simulink model "KinarmUAATask_260120"  (R2019b)
settings: Solver=ode4  StartTime=0.0  StopTime=inf  FixedStep=BKIN_STEP_TIME  RelTol=1e-3  EnableMultiTasking=on
StartFcn:
  |  warndlg('Dexterit-E models cannot run under simulation. Please compile your model and run it from within Dexterit-E.');set_param(bdroot,'SimulationCommand','stop')
model workspace (MAT data in the model file):
  APPROACH_TARGET_COL = 6
  AVOID_TARGET_COL = 2
  BEGIN_TARGET_COL = 3
  BKIN_KINEMATIC_FRAME_SIZE = 400
  BKIN_STEP_TIME = 0.00025
  COLOUR_2ND = 7
  COLOUR_3RD = 11
  COLOUR_4TH = 12
  COLOUR_INIT = 6
  E_APPROACHED = 25
  E_AVOIDED = 23
  E_COND1_APP = 24
  E_COND2_APP = 18
  E_ERROR_TRIAL = 21
  E_FALSE_START = 16
  E_HAND_IN_START = 15
  E_LOC_1 = 1
  E_LOC_10 = 10
  E_LOC_11 = 11
  E_LOC_12 = 12
  E_LOC_2 = 2
  E_LOC_3 = 3
  E_LOC_4 = 4
  E_LOC_5 = 5
  E_LOC_6 = 6
  E_LOC_7 = 7
  E_LOC_8 = 8
  E_LOC_9 = 9
  E_NEUT1_APP = 22
  E_NEUT2_APP = 17
  E_NO_EVENT = 0
  E_SUCCESS_TRIAL = 26
  E_TARGET_ON = 14
  E_TIMED_OUT = 20
  E_TRIAL_COND1 = 27
  E_TRIAL_COND2 = 28
  E_TRIAL_END = 19
  E_TRIAL_NEUT1 = 29
  E_TRIAL_NEUT2 = 30
  E_TRIAL_START = 13
  INFO_TARGET_COL = 5
  LABEL_COL = 4
  LABEL_HEIGHT = 9
  LABEL_TEXT = 8
  LENGTH = 3
  MAX_FORCE = 2
  NEUT_OR_COND = 7
  NUM_SPOTS = 8
  POSTRESP_DELAY = 7
  RADIUS_VIS = 3
  RAMP_DURATION = 3
  REACH_DELAY = 4
  REACH_RAND = 5
  REACH_TO = 6
  START_BLOCK = 9
  START_TARGET_COL = 1
  STROKE_WIDTH = 10
  TARGET_X = 4
  TARGET_Y = 5
  TARG_DIST = 1
  TARG_LENGTH = 3
  TARG_WIDTH = 4
  TOGGLE_FIELD = 8
  WIDTH = 4
  Width = 4
  col_x = 1
  col_y = 2
undefined symbols (not defined in the file or in its folder): slselsubs
libraries: Video x7, General x3, KINARM_general x2, KINARM_EP_loads x2
settings Model: ModifiedComment=chris -- Wed Feb 16 09:18:30 2005 -- Version 1.1384  ModifiedHistory=Feb 16/05 - Add error repeat, add offset ramp  ExtModeArmWhenConnect=off  ExtModeLogAll=off  OrderedModelArguments=off  Creator=Chris Grebeldinger  LastModifiedBy=apark2
settings SolverCC: AutoInsertRateTranBlk=on
settings DataIOCC: SaveFormat=Array  SignalLoggingSaveFormat=ModelDataLogs  SaveOutput=off  SaveTime=off  ReturnWorkspaceOutputs=off  SignalLoggingName=sigsOut
settings OptimizationCC: BlockReduction=off  BooleanDataType=off  OptimizeBlockIOStorage=off  BufferReuse=off  GlobalBufferReuse=off  ExpressionFolding=off  ExpressionDepthLimit=2147483647  LocalBlockOutputs=off  InitFltsAndDblsToZero=on  LifeSpan=inf  OptimizeDataStoreBuffers=off  BusAssignmentInplaceUpdate=off
settings DebuggingCC: SaveWithParameterizedLinksMsg=none  UnderspecifiedInitializationDetection=Classic  MergeDetectMultiDrivingBlocksExec=none  SignalResolutionControl=TryResolveAllWithWarning  MultiTaskDSMMsg=warning  FcnCallInpInsideContextMsg=warning  BusObjectLabelMismatch=none  StateNameClashWarn=warning  StrictBusMsg=ErrorOnBusTreatedAsVector  SFUnexpectedBacktrackingDiag=warning  SFNoUnconditionalDefaultTransitionDiag=warning  SFExecutionAtInitializationDiag=none  ArithmeticOperatorsInVariantConditions=warning
settings HardwareCC: ProdBitPerPointer=32  ProdBitPerSizeT=32  ProdBitPerPtrDiffT=32  ProdLargestAtomicFloat=None  ProdWordSize=32  ProdLongLongMode=on  ProdHWDeviceType=Generic->32-bit x86 compatible  TargetLongLongMode=on  TargetIntDivRoundTo=Zero  TargetEndianess=LittleEndian  TargetHWDeviceType=Generic->32-bit x86 compatible
settings ModelReferenceCC: PropagateSignalLabelsOutOfModel=off
settings SFSimCC: SimCustomHeaderCode="#include \"stdlib.h\""  SimUseLocalCustomCode=off  SimParseCustomCode=off  CustomCodeUndefinedFunction=UseInterfaceOnly
settings RTWCC: Description=Simulink Real-Time  SystemTargetFile=slrt.tlc  TemplateMakefile=slrt_default_tmf  RTWUseLocalCustomCode=off  CustomSourceCode="#include \"stdlib.h\""  CodeExecutionProfiling=on
settings CodeAppCC: MaxIdLength=63  StateflowObjectComments=on
settings SimulinkRealTimeCC: TargetFcnLib=ansi_tfl_tmw.mat  GeneratePreprocessorConditionals=Disable all  PreserveStateflowLocalDataDimensions=off
settings ConfigComp: CovMetricSettings=dw  CovHtmlReporting=on  CovSaveCumulativeToWorkspaceVar=on  CovSaveSingleToWorkspaceVar=on  CovExternalEMLEnable=off

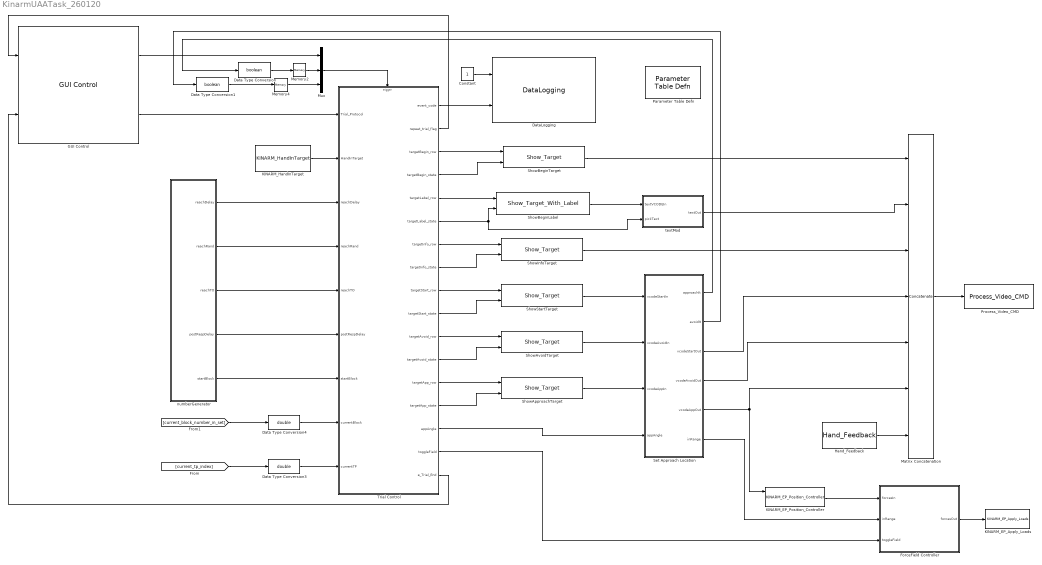
== system KinarmUAATask_260120 ==
  Constant : Constant
  Data Type Conversion : DataTypeConversion  OutDataTypeStr=boolean
  Data Type Conversion1 : DataTypeConversion  OutDataTypeStr=boolean
  Data Type Conversion3 : DataTypeConversion  OutDataTypeStr=double
  Data Type Conversion4 : DataTypeConversion  OutDataTypeStr=double
  DataLogging : General/DataLogging  log_event_codes=on  log_analog_inputs=off  show_time_remaining=off  ecat_include=on
  ForceField Controller : Subsystem
  GUI Control : General/GUI Control  task_version=1.0  show_repeat_trial_flag=on  use_custom_tp=off  target_type_str=Circle  Target_Type=1  XYcols=[1 2]  Vcols=3  Lcols=4  indices_padding=[0 0 0 0;0 0 0 0]  target_table_rows=64  load_table_rows=20  tp_table_rows=100
  Hand_Feedback : KINARM_general/Hand_Feedback  feedback_cntl_src=none
  KINARM_EP_Apply_Loads : KINARM_EP_loads/KINARM_EP_Apply_Loads  up_duration=1500  down_duration=1500  max_force=30
  KINARM_EP_Position_Controller : KINARM_EP_loads/KINARM_EP_Position_Controller  use_dom_hand=on  inertias_for_FF=KINARM End Point robot  gain_choice=Standard Movement  sample_time=0.001
  KINARM_HandInTarget : KINARM_general/KINARM_HandInTarget  use_dominant_hand=on  target_type=Circle  num_states=1  attribcol1=[RADIUS_VIS]  attribcol2=[0]  attribcol3=[0]  attribcol4=[0]  attribcol5=[0]
  Matrix Concatenation : Concatenate  NumInputs=7  Mode=Multidimensional array
  Memory2 : Memory
  Memory4 : Memory
  Mux : Mux  Inputs=3
  Parameter Table Defn : General/Parameter Table Defn  ShowInLibBrowser=0
  Process_Video_CMD : Video/Process_Video_CMD  video_delay=50
  Set Approach Location : Subsystem
  ShowApproachTarget : Video/Show_Target  target_type=Circle  num_states=1  attribcol1=[COLOUR_INIT 0 0 RADIUS_VIS]  attribcol2=[0 0 0 0]  attribcol3=[0 0 0 0]  attribcol4=[0 0 0 0]  attribcol5=[0 0 0 0]  stateindices_padding=[0 0 0 0 0 0 0;0 0 0 0 0 0 0;0 0 0 0 0 0 0;0 0 0 0 0 0 0;0 0 0 0 0 0 0]  source=dialog  opacity=100  target_display=Both subject and operator displays  num_col=4
  ShowAvoidTarget : Video/Show_Target  target_type=Circle  num_states=1  attribcol1=[COLOUR_INIT COLOUR_2ND STROKE_WIDTH RADIUS_VIS]  attribcol2=[0 0 0 0]  attribcol3=[0 0 0 0]  attribcol4=[0 0 0 0]  attribcol5=[0 0 0 0]  stateindices_padding=[0 0 0 0 0 0 0;0 0 0 0 0 0 0;0 0 0 0 0 0 0;0 0 0 0 0 0 0;0 0 0 0 0 0 0]  source=dialog  opacity=100  target_display=Both subject and operator displays  num_col=4
  ShowBeginLabel : Video/Show_Target_With_Label  target_type=Circle  num_states=3  attribcol1=[0 0 0 0 LABEL_TEXT COLOUR_INIT LABEL_HEIGHT]  attribcol2=[0 0 0 0 LABEL_TEXT COLOUR_2ND LABEL_HEIGHT]  attribcol3=[0 0 0 0 LABEL_TEXT COLOUR_3RD LABEL_HEIGHT]  attribcol4=[0 0 0 0 0 0 0]  attribcol5=[0 0 0 0 0 0 0]  stateindices_padding=[0 0 0 0;0 0 0 0;0 0 0 0;0 0 0 0;0 0 0 0]  source=dialog  opacity=100  target_display=Both subject and operator displays
  ShowBeginTarget : Video/Show_Target  target_type=Circle  num_states=1  attribcol1=[COLOUR_INIT COLOUR_2ND STROKE_WIDTH RADIUS_VIS]  attribcol2=[0 0 0 0]  attribcol3=[0 0 0 0]  attribcol4=[0 0 0 0]  attribcol5=[0 0 0 0]  stateindices_padding=[0 0 0 0 0 0 0;0 0 0 0 0 0 0;0 0 0 0 0 0 0;0 0 0 0 0 0 0;0 0 0 0 0 0 0]  source=dialog  opacity=100  target_display=Both subject and operator displays  num_col=4
  ShowInfoTarget : Video/Show_Target  target_type=Rectangle  num_states=4  attribcol1=[COLOUR_INIT 0 0 TARGET_X TARGET_Y 0]  attribcol2=[COLOUR_2ND 0 0 TARGET_X TARGET_Y 0]  attribcol3=[COLOUR_3RD 0 0 TARGET_X TARGET_Y 0]  attribcol4=[COLOUR_4TH 0 0 TARGET_X TARGET_Y 0]  attribcol5=[0 0 0 0 0 0]  stateindices_padding=[0 0 0 0 0;0 0 0 0 0;0 0 0 0 0;0 0 0 0 0;0 0 0 0 0]  source=dialog  opacity=100  target_display=Both subject and operator displays  num_col=6
  ShowStartTarget : Video/Show_Target  target_type=Circle  num_states=1  attribcol1=[COLOUR_INIT COLOUR_2ND STROKE_WIDTH RADIUS_VIS]  attribcol2=[0 0 0 0]  attribcol3=[0 0 0 0]  attribcol4=[0 0 0 0]  attribcol5=[0 0 0 0]  stateindices_padding=[0 0 0 0 0 0 0;0 0 0 0 0 0 0;0 0 0 0 0 0 0;0 0 0 0 0 0 0;0 0 0 0 0 0 0]  source=dialog  opacity=100  target_display=Both subject and operator displays  num_col=4
  Trial Control : Stateflow chart  TreatAsAtomicUnit=on
  numberGenerator : Subsystem
  textMod : Subsystem
  wires:
  Trial Control/17(e_Trial_End) -> GUI Control/2
  Trial Control/10(targetStart_state) -> ShowStartTarget/2
  Trial Control/9(targetStart_row) -> ShowStartTarget/1
  Matrix Concatenation/1 -> Process_Video_CMD/1
  Trial Control/1(event_code) -> DataLogging/2
  ShowStartTarget/1 -> Set Approach Location/1(vcodeStartIn)
  Constant/1 -> DataLogging/1
  GUI Control/2 -> Trial Control/1(Trial_Protocol)
  Trial Control/13(targetApp_row) -> ShowApproachTarget/1
  Trial Control/14(targetApp_state) -> ShowApproachTarget/2
  Trial Control/2(repeat_trial_flag) -> GUI Control/1
  KINARM_EP_Position_Controller/1 -> ForceField Controller/1(forcesIn)
  [current_tp_index] -> Data Type Conversion3/1
  ShowApproachTarget/1 -> Set Approach Location/3(vcodeAppIn)
  Set Approach Location/5(vcodeAppOut) -> Matrix Concatenation/6, KINARM_EP_Position_Controller/1
  Trial Control/15(appAngle) -> Set Approach Location/4(appAngle)
  ShowInfoTarget/1 -> Matrix Concatenation/3
  KINARM_HandInTarget/1 -> Trial Control/2(HandInTarget)
  Trial Control/16(toggleField) -> ForceField Controller/3(toggleField)
  ForceField Controller/1(forcesOut) -> KINARM_EP_Apply_Loads/1
  Trial Control/3(targetBegin_row) -> ShowBeginTarget/1
  Trial Control/4(targetBegin_state) -> ShowBeginTarget/2
  Trial Control/7(targetInfo_row) -> ShowInfoTarget/1
  Trial Control/8(targetInfo_state) -> ShowInfoTarget/2
  Trial Control/5(targetLabel_row) -> ShowBeginLabel/1
  Trial Control/6(targetLabel_state) -> ShowBeginLabel/2, textMod/2(pickText)
  numberGenerator/1(reachDelay) -> Trial Control/3(reachDelay)
  numberGenerator/2(reachRand) -> Trial Control/4(reachRand)
  numberGenerator/3(reachTO) -> Trial Control/5(reachTO)
  numberGenerator/4(postRespDelay) -> Trial Control/6(postRespDelay)
  ShowBeginLabel/1 -> textMod/1(textVCODEIn)
  ShowBeginTarget/1 -> Matrix Concatenation/1
  Hand_Feedback/1 -> Matrix Concatenation/7
  Set Approach Location/6(inRange) -> ForceField Controller/2(inRange)
  Data Type Conversion3/1 -> Trial Control/9(currentTP)
  Trial Control/11(targetAvoid_row) -> ShowAvoidTarget/1
  Trial Control/12(targetAvoid_state) -> ShowAvoidTarget/2
  ShowAvoidTarget/1 -> Set Approach Location/2(vcodeAvoidIn)
  [current_block_number_in_set] -> Data Type Conversion4/1
  Data Type Conversion4/1 -> Trial Control/8(currentBlock)
  textMod/1(textOut) -> Matrix Concatenation/2
  Data Type Conversion1/1 -> Memory4/1
  Memory4/1 -> Mux/3
  Data Type Conversion/1 -> Memory2/1
  Memory2/1 -> Mux/2
  Mux/1 -> Trial Control/Trigger
  GUI Control/1 -> Mux/1
  Set Approach Location/1(approachIt) -> Data Type Conversion/1
  Set Approach Location/4(vcodeAvoidOut) -> Matrix Concatenation/5
  Set Approach Location/2(avoidIt) -> Data Type Conversion1/1
  Set Approach Location/3(vcodeStartOut) -> Matrix Concatenation/4
  numberGenerator/5(startBlock) -> Trial Control/7(startBlock)

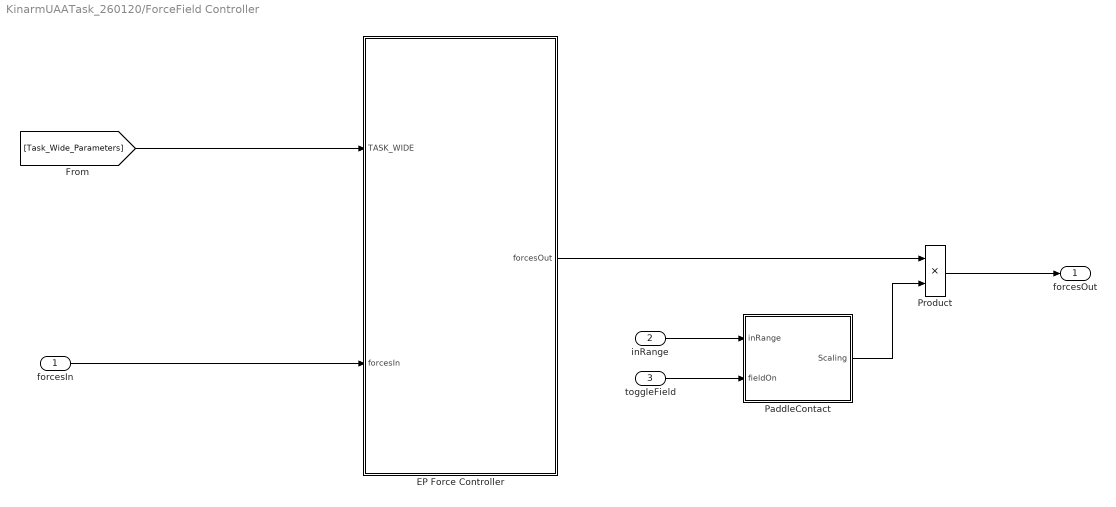
== system KinarmUAATask_260120/ForceField Controller ==
  forcesIn : Inport
  inRange : Inport  Port=2
  toggleField : Inport  Port=3
  EP Force Controller : MATLAB Function  TreatAsAtomicUnit=on
  PaddleContact : Subsystem  mask(Perturbation){}
  Product : Product
  forcesOut : Outport
  wires:
  [Task_Wide_Parameters] -> EP Force Controller/1(TASK_WIDE)
  EP Force Controller/1(forcesOut) -> Product/1
  toggleField/1 -> PaddleContact/2(fieldOn)
  forcesIn/1 -> EP Force Controller/2(forcesIn)
  PaddleContact/1(Scaling) -> Product/2
  inRange/1 -> PaddleContact/1(inRange)
  Product/1 -> forcesOut/1

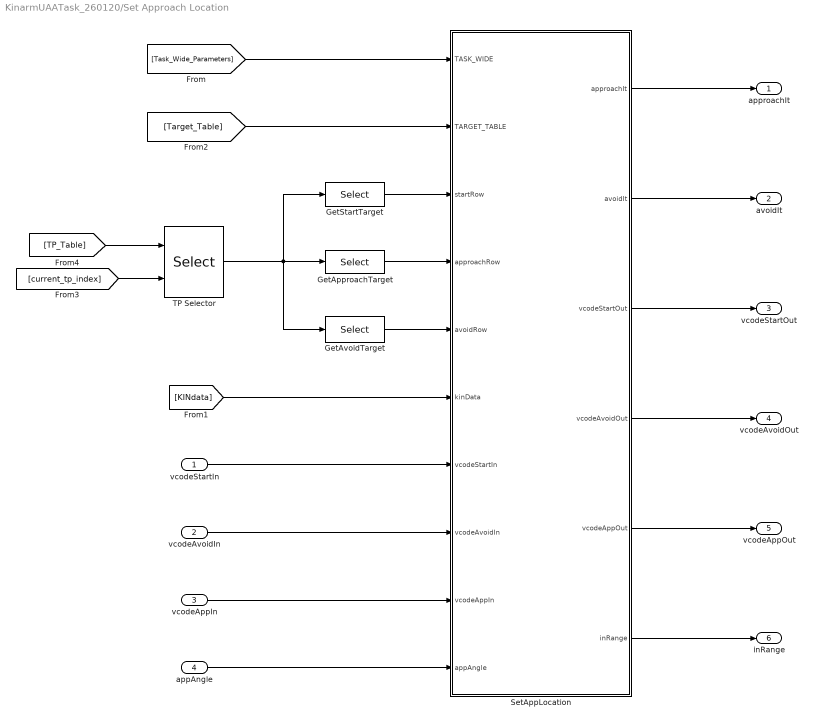
== system KinarmUAATask_260120/Set Approach Location ==
  vcodeStartIn : Inport
  vcodeAvoidIn : Inport  Port=2
  vcodeAppIn : Inport  Port=3
  appAngle : Inport  Port=4
  GetApproachTarget : Selector  NumberOfDimensions=2  InputPortWidth=3  IndexOptions=Select all,Index vector (dialog)  Indices=[1],[APPROACH_TARGET_COL]  OutputSizes=slselsubs([(-2),(-2)],1),slselsubs([(-2),(-2)],2)
  GetAvoidTarget : Selector  NumberOfDimensions=2  InputPortWidth=3  IndexOptions=Select all,Index vector (dialog)  Indices=[1],[AVOID_TARGET_COL]  OutputSizes=slselsubs([(-2),(-2)],1),slselsubs([(-2),(-2)],2)
  GetStartTarget : Selector  NumberOfDimensions=2  InputPortWidth=3  IndexOptions=Select all,Index vector (dialog)  Indices=[1],[START_TARGET_COL]  OutputSizes=slselsubs([(-2),(-2)],1),slselsubs([(-2),(-2)],2)
  SetAppLocation : MATLAB Function  TreatAsAtomicUnit=on
  TP Selector : Selector  NumberOfDimensions=2  InputPortWidth=3  IndexOptions=Index vector (port),Select all  Indices=1,-1  OutputSizes=slselsubs([(-2),(-2)],1),slselsubs([(-2),(-2)],2)
  approachIt : Outport
  avoidIt : Outport  Port=2
  vcodeStartOut : Outport  Port=3
  vcodeAvoidOut : Outport  Port=4
  vcodeAppOut : Outport  Port=5
  inRange : Outport  Port=6
  wires:
  [Task_Wide_Parameters] -> SetAppLocation/1(TASK_WIDE)
  [current_tp_index] -> TP Selector/2
  [KINdata] -> SetAppLocation/6(kinData)
  [TP_Table] -> TP Selector/1
  [Target_Table] -> SetAppLocation/2(TARGET_TABLE)
  vcodeAppIn/1 -> SetAppLocation/9(vcodeAppIn)
  SetAppLocation/5(vcodeAppOut) -> vcodeAppOut/1
  GetStartTarget/1 -> SetAppLocation/3(startRow)
  appAngle/1 -> SetAppLocation/10(appAngle)
  SetAppLocation/6(inRange) -> inRange/1
  vcodeAvoidIn/1 -> SetAppLocation/8(vcodeAvoidIn)
  GetAvoidTarget/1 -> SetAppLocation/5(avoidRow)
  GetApproachTarget/1 -> SetAppLocation/4(approachRow)
  TP Selector/1 -> GetStartTarget/1, GetAvoidTarget/1, GetApproachTarget/1
  SetAppLocation/4(vcodeAvoidOut) -> vcodeAvoidOut/1
  SetAppLocation/1(approachIt) -> approachIt/1
  SetAppLocation/2(avoidIt) -> avoidIt/1
  vcodeStartIn/1 -> SetAppLocation/7(vcodeStartIn)
  SetAppLocation/3(vcodeStartOut) -> vcodeStartOut/1

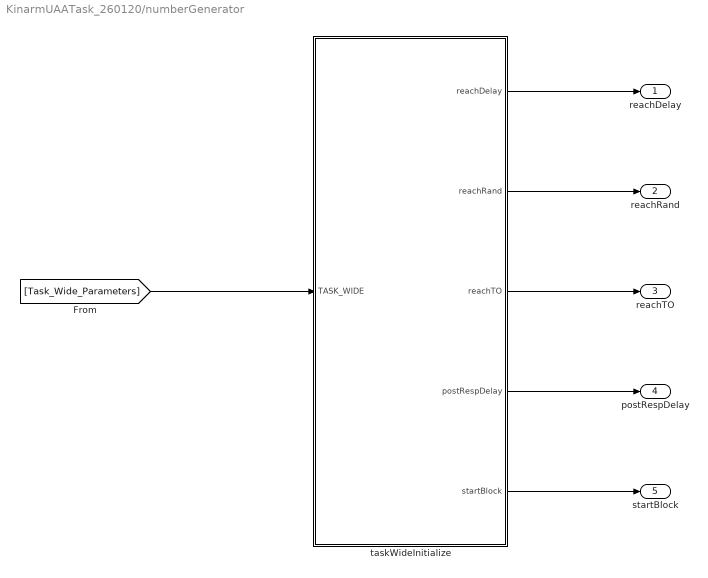
== system KinarmUAATask_260120/numberGenerator ==
  taskWideInitialize : MATLAB Function  TreatAsAtomicUnit=on
  reachDelay : Outport
  reachRand : Outport  Port=2
  reachTO : Outport  Port=3
  postRespDelay : Outport  Port=4
  startBlock : Outport  Port=5
  wires:
  [Task_Wide_Parameters] -> taskWideInitialize/1(TASK_WIDE)
  taskWideInitialize/1(reachDelay) -> reachDelay/1
  taskWideInitialize/2(reachRand) -> reachRand/1
  taskWideInitialize/3(reachTO) -> reachTO/1
  taskWideInitialize/4(postRespDelay) -> postRespDelay/1
  taskWideInitialize/5(startBlock) -> startBlock/1

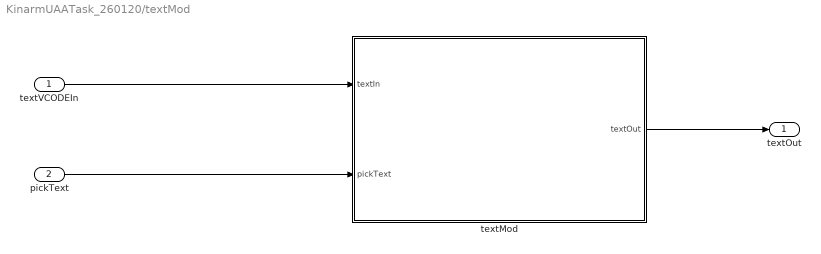
== system KinarmUAATask_260120/textMod ==
  textVCODEIn : Inport
  pickText : Inport  Port=2
  textMod : MATLAB Function  TreatAsAtomicUnit=on
  textOut : Outport
  wires:
  textMod/1(textOut) -> textOut/1
  textVCODEIn/1 -> textMod/1(textIn)
  pickText/1 -> textMod/2(pickText)

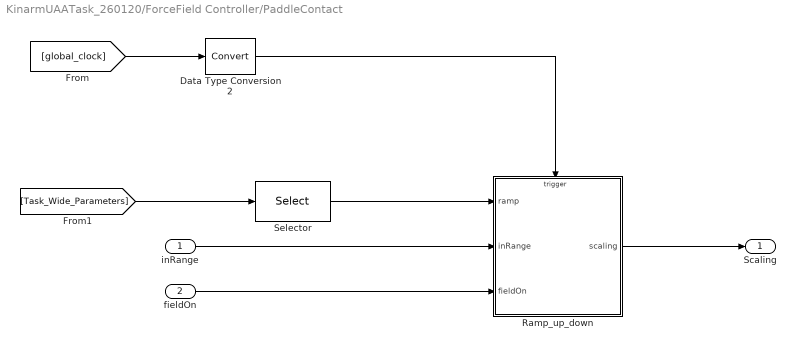
== system KinarmUAATask_260120/ForceField Controller/PaddleContact ==
  inRange : Inport
  fieldOn : Inport  Port=2
  Data Type Conversion2 : DataTypeConversion
  Ramp_up_down : Stateflow chart  TreatAsAtomicUnit=on
  Selector : Selector  NumberOfDimensions=2  InputPortWidth=3  IndexOptions=Index vector (dialog),Select all  Indices=[RAMP_DURATION],[3]  OutputSizes=slselsubs([(-2),(-2)],1),1
  Scaling : Outport
  wires:
  Ramp_up_down/1(scaling) -> Scaling/1
  [global_clock] -> Data Type Conversion2/1
  Data Type Conversion2/1 -> Ramp_up_down/Trigger
  [Task_Wide_Parameters] -> Selector/1
  Selector/1 -> Ramp_up_down/1(ramp)
  inRange/1 -> Ramp_up_down/2(inRange)
  fieldOn/1 -> Ramp_up_down/3(fieldOn)

== matlab function KinarmUAATask_260120/Set Approach Location/SetAppLocation ==
  data: approachIt output; avoidIt output; vcodeStartOut output; vcodeAvoidOut output; vcodeAppOut output; TASK_WIDE input; TARGET_TABLE input; startRow input; approachRow input; avoidRow input; kinData input; vcodeStartIn input; vcodeAvoidIn input; vcodeAppIn input; appAngle input; TARG_DIST parameter; RADIUS_VIS parameter; inRange output; NUM_SPOTS parameter
function [approachIt, avoidIt, vcodeStartOut, vcodeAvoidOut, vcodeAppOut, inRange] = fcn...
    (TASK_WIDE, TARGET_TABLE, startRow, approachRow, avoidRow, kinData, vcodeStartIn, vcodeAvoidIn, vcodeAppIn, appAngle,...
    TARG_DIST, RADIUS_VIS, NUM_SPOTS)
%This function checks if the hand is in the approach or avoid targets and passing through the start target for nice visuals.

%% initialize hand and location to be displayed
targDist = TASK_WIDE(TARG_DIST)*0.01; %gets distance of targets set from task wide
numSpots = TASK_WIDE(NUM_SPOTS); %get the number of reach spots but still needs a change in the Trial Control to align with the maximum appAngle
angleArray = [0:2*pi/numSpots:2*pi-2*pi/numSpots]; %get radians for each location

whichLoc = angleArray(appAngle); %get the location

%% initialize radius
vcodeStartOut = vcodeStartIn; %start target routed through this function
rValStart = TARGET_TABLE(startRow,RADIUS_VIS)*0.01; %radius of start target
rValApp = TARGET_TABLE(approachRow,RADIUS_VIS)*0.01; %radius of approach target
rValApp2 = targDist-rValStart; %radius of force field around approach target accounts for starting target
rValAvoid = TARGET_TABLE(avoidRow,RADIUS_VIS)*0.01; %radius of avoid target

asseHand=kinData(3,1); %check which hand is used
handX = kinData(asseHand,23); %get the x position of the hand
handY = kinData(asseHand,24); %get the y position of the hand

%% change vcodes for approach target contact
%Rip off of handintarget function for a shifted approach target (circle).
vcodeAppOut = vcodeAppIn;

vcodeAppOut(3) = vcodeStartIn(3) + targDist*cos(whichLoc); %get shifted x position of the approach target
vcodeAppOut(4) = vcodeStartIn(4) + targDist*sin(whichLoc); %get shifted y position of the approach target

deltaxApp=handX-vcodeAppOut(3); %get the difference between hand x position and approach target x position
deltayApp=handY-vcodeAppOut(4); %get the difference between hand y position and approach target y position

distanceApp = deltaxApp.^2 + deltayApp.^2; %get the hypotenuse squared
if (distanceApp < rValApp^2) %if hand inside approach target
    approachIt = 1; %flag is 1
else
    approachIt = 0; %flag is 0
end

%if hand inside the force field, won't turn on forcefield unless
%toggleField = 1 in Trial Control
if (distanceApp < rValApp2^2) %check if hand is within forcefield
    inRange = 1; %flag is 1
else
    inRange = 0; %flag is 0
end

%% change vcodes for avoid target no contact
%similar to above but checks if hand is inside avoid target (circle)

vcodeAvoidOut = vcodeAvoidIn;

vcodeAvoidOut(3) = vcodeStartIn(3) + targDist*cos(whichLoc+pi); %shifted x position of avoid target
vcodeAvoidOut(4) = vcodeStartIn(4) + targDist*sin(whichLoc+pi);

deltaxAvoid=handX-vcodeAvoidOut(3);
deltayAvoid=handY-vcodeAvoidOut(4);

distanceAvoid = deltaxAvoid.^2 + deltayAvoid.^2;
if (distanceAvoid < rValAvoid^2) %if hand inside approach target
    avoidIt = 1;
else
    avoidIt = 0;
end

== stateflow chart KinarmUAATask_260120/Trial Control ==
  note: ************************Preface***************************:
      | The UKA task examines approach and avoidance tendencies to certain visual stimulus shown to participants. Typically, two conditions are used and testing by having participants remember
      | to approach one condition and avoid the other (move in the opposite direction). This is done in one block and the association is reverse in the next block.
      | Previous approach and avoidance tasks AAT used keyboard presses or joysticks to examine these tendencies but were biased by testing only unimanual movements.
      |
      | This adaptation of the AAT examines tendencies in 12 different directions where 1 is east of the start target, 4 is north, 7 is west, and 10 is south.
      | This version has neutral conditions that compares baseline movements to neutral stimulus resulting in 4 different types of images.
      | The current .dtp file uses 6 different images of condition1 and 6 images of condition2 stimulus and 6 neutral images based on the shape of the condition1 images and 6 neutral images
      | based on the shape of the condition2 images. Each image is associated with a specific TP so there are 24 total TP to call. TP1-6 are condition1 images, 7-12 are condition2 images,
      | 13-18 are neutral condition1 images, 19-24 are neutral condition2 images.
      |
      | The task is set up so that each block only consists of conditions or neutral images so each block has only TP1-12 or TP13-24. In each of these blocks, each condition or neutral image
      | appears in each of the 12 directions at least once (i.e. in a condition block, TP1-6 appears in locations 1-12 at least once and TP7-12 appears at least once so each set of 6TP needs
      | to be run twice as a group of 24 trials for an even distribution of conditions/reach direction).
      |
      | The task must be run in 4 blocks starting and ending with a condition or neutral block, and the middle two blocks being the other block type for proper task operation. The UKA
      | randomly selects which condition will first be associated with approach and avoidance but when the next block of the same condition appears, the association is automatically
      | reversed (neutCount == 1 or condCount == 1).
      |
      | *This layout assumes the task has 12 directions of reach and 6images per 4conditions to run properly
      | *Modifying the task to have less reach directions, less images in the TP, or a different number of blocks requires testing
      | *approaching a condition also equals avoiding the other within each block
  state Initialize/
    %set up targets and states
    entry:
    targetInfo_row = Trial_Protocol(INFO_TARGET_COL); %image of approach/avoid association
    targetBegin_row = Trial_Protocol(BEGIN_TARGET_COL); %block start target
    targetStart_row = Trial_Protocol(START_TARGET_COL); %trial start target
    targetApp_row = Trial_Protocol(APPROACH_TARGET_COL); %approach target
    targetAvoid_row = Trial_Protocol(AVOID_TARGET_COL); %avoid target
    targetLabel_row = Trial_Protocol(LABEL_COL); %target for displaying text
    targetInfo_state = 0; %turn off information target
    targetBegin_state = 0; %turn off block start trial
    targetStart_state = 0; %turn off trial start target
    targetApp_state = 0; %turn off approach target
    targetAvoid_state = 0; %turn off avoid target
    targetLabel_state = 0; %turn off label
  state MainTrial/
    state StartofTrial/
      %start trial
      entry:
      targetApp_row = Trial_Protocol(APPROACH_TARGET_COL); %approach target
      targetAvoid_row = Trial_Protocol(AVOID_TARGET_COL); %avoid target
      randReach = reachRand*rand(); %get random value for reachRand
      targetStart_state = 1; %show start trial target
      targetApp_state = 0; %turn off approach target
      targetAvoid_state = 0; %turn off avoid target
      toggleField = 0; %no forcefield also doubles as indicating cond2/neut2 targets
      targetBegin_state = 0; %turn off start task target
      targetLabel_state = 0; %turn off labels
      targetInfo_state = 0; %turn off info target
      countTP(currentTP) = countTP(currentTP) + 1; %increment the countTP at the currentTP index
      [appAngle, condNeut] = arraySets(randA,randB,countTP,currentTP); %function to get random location
      event_code = E_TRIAL_START; %trial started
    state condEvents/
      state approachCond1/
        event_code = E_COND1_APP;
        targetInfo_state = 1; %turn on info
      state approachCond2/
        event_code = E_COND2_APP;
        targetInfo_state = 2; %turn on info
    state waitForHold/
    state outputBlockOrder/
      %set up approach or avoid for condition and neutral trials based on even or odd of the current trial
      entry:
      appAvoidCond = mod(currentTP,2); %even is approach cond1/avoid cond2, odd is approach cond2/avoid cond1
      appAvoidNeut = mod(currentTP,2); %same as condition block
      condCount = 0; %count the condition blocks
      neutCount = 0; %count the neutral blocks
    state condCount/
      %sets the condition block
      entry:
      condCount = condCount + 1; %increment condition block
      appAvoid = appAvoidCond; %set approach/avoid
    state blockStart/
      %get the current block number and set up TP counter
      %and randA for random order for cond1/neut1 and
      %randB for cont2/neut2. Not sure how to make
      %randperm take Task_Wide input
      entry:
      blockCheck = currentBlock; %update blockNumber
      targetBegin_state = 1; %turn on task start target
      targetLabel_state = 1; %turn on label target
      countTP = zeros(1,24); %set TP count
      randA = randperm(12); %set rand array of locations
      randB = randperm(12); %set rand array of locations
    state handStart/
      %participant reads
      %instructions so wait for
      %the hand to be in start
      %target for some time
    state left/
      %event code for hand leaving start
      event_code = E_FALSE_START;
    state AppOn/
      %turn on targets for reaching
      entry:
      toggleField = Trial_Protocol(TOGGLE_FIELD); %check if trial
      %has forcefield turns on a forcefield if it is set but also just
      %indicates that a trial is cond1/neut1 (1) or cond2/neut2 (2)
      targetStart_state = 0; %turn off start target
      targetApp_state = 1; %turn on approach target
      targetAvoid_state = 1; %turn on avoid target
    state swapNeutBlock/
      %swap the approach avoid rule
      entry:
      appAvoidNeut = 1-appAvoidNeut;
    state neutCount/
      %sets the neutral block
      entry:
      neutCount = neutCount + 1; %increment neutral block
      appAvoid = appAvoidNeut; %set approach from current block type
    state whichSide/
      %the hand is in the start target
      event_code = E_HAND_IN_START;
    state conditionEvents
      state eventCond1/
        event_code = E_TRIAL_COND1;
      state eventCond2/
        event_code = E_TRIAL_COND2;
      state eventNeut1/
        event_code = E_TRIAL_NEUT1;
      state eventNeut2/
        event_code = E_TRIAL_NEUT2;
    state swapCondBlock/
      %swap the approach avoid condition
      entry:
      appAvoidCond = 1-appAvoidCond;
    state neutEvents/
      state approachNeut1/
        event_code = E_NEUT1_APP;
        targetInfo_state = 3; %turn on info
      state approachNeut2/
        event_code = E_NEUT2_APP;
        targetInfo_state = 4; %turn on info
    state nice1/
    state waitForHold1/
    state nice/
    state Approached/
      %hand is in approach
      event_code = E_APPROACHED;
      toggleField = 0; %turn off forcefield
    state locationEvents/
      state loc1/
        event_code = E_LOC_1;
      state loc2/
        event_code = E_LOC_2;
      state loc3/
        event_code = E_LOC_3;
      state loc4/
        event_code = E_LOC_4;
      state loc5/
        event_code = E_LOC_5;
      state loc6/
        event_code = E_LOC_6;
      state loc7/
        event_code = E_LOC_7;
      state loc8/
        event_code = E_LOC_8;
      state loc9/
        event_code = E_LOC_9;
      state loc10/
        event_code = E_LOC_10;
      state loc11/
        event_code = E_LOC_11;
      state loc12/
        event_code = E_LOC_12;
    state checkError/
      %trial was error
      event_code = E_ERROR_TRIAL;
      targetLabel_state = 2; %incorrect!
    state Avoided/
      %hand left avoid target
      event_code = E_AVOIDED;
      toggleField = 0; %turn off forcefield
    state success/
      %trial was successful
      event_code = E_SUCCESS_TRIAL;
    state EndOfTrial/
      % Turn off targets,
      targetStart_state = 0; %turn off start target
      targetAvoid_state = 0; %turn off avoid target
      targetApp_state = 0; %turn off approach target
      toggleField = 0; %turn off forcefield
    state TimedOut/
      %too slow to reach start/app/avoid
      event_code = E_TIMED_OUT;
      targetLabel_state = 3; %too slow!
      toggleField = 0; %turn off forcefield
    condEvents -> waitForHold : after(1,msec)
    condCount -> approachCond1 [order 1] : %approach cond1
        | [appAvoid == 0]
    waitForHold -> handStart : %hand in
        | [HandInTarget(targetBegin_row) == 1]
    handStart -> waitForHold [order 2] : %hand out
        | [HandInTarget(targetBegin_row) == 0]
    (junction 357) -> outputBlockOrder [order 2] : %if second neut block finished
        | [neutCount == 2]
    (junction 355) -> outputBlockOrder [order 2] : %if second cond block finished
        | [condCount == 2]
    outputBlockOrder -> blockStart : %start task
    condCount -> approachCond2 [order 2] : %approach cond2
        | [appAvoid == 1]
    handStart -> StartofTrial [order 3] : %hand in start target for long enough
        | after(startBlock,msec)
    StartofTrial -> (junction 455)
    blockStart -> condCount [order 1] : %if condition block
        | [Trial_Protocol(NEUT_OR_COND) == 1]
    (junction 357) -> blockStart [order 1] : %if no neut block started
        | [neutCount == 0]
    (junction 357) -> swapNeutBlock [order 3] : %if first neut block finished
        | [neutCount == 1]
    waitForHold1 -> handStart : %hand in
        | [HandInTarget(targetBegin_row) == 1]
    handStart -> waitForHold1 [order 1] : %hand out
        | [HandInTarget(targetBegin_row) == 0]
    (junction 323) -> (junction 357) [order 2] : %if neutral block
        | [Trial_Protocol(NEUT_OR_COND) == 0]
    left -> (junction 455) : %after a time
        | after(postRespDelay/2,msec)
    (junction 455) -> whichSide : %checks if hand is in start
        | [HandInTarget(targetStart_row) == 1]
    whichSide -> left [order 1] : %check if hand left start
        | [HandInTarget(targetStart_row) == 0]
    blockStart -> neutCount [order 2] : %if neutral block
        | [Trial_Protocol(NEUT_OR_COND) == 0]
    swapNeutBlock -> blockStart
    (junction 355) -> blockStart [order 1] : %if no cond block started
        | [condCount == 0]
    swapCondBlock -> blockStart
    whichSide -> AppOn [order 2] : %hand in start delay
        | after(reachDelay+randReach,msec)
    neutCount -> approachNeut2 [order 1] : %approach neut2
        | [appAvoid == 1]
    neutCount -> approachNeut1 [order 2] : %approach neut1
        | [appAvoid == 0]
    AppOn -> eventCond1 [order 2] : %condition1
        | [condNeut == 1]
    AppOn -> eventCond2 [order 3] : %condition 2
        | [condNeut == 2]
    AppOn -> eventNeut1 [order 4] : %neutral 1
        | [condNeut == 3]
    AppOn -> eventNeut2 [order 1] : %neutral 2
        | [condNeut == 4]
    (junction 323) -> (junction 355) [order 1] : %if condition block
        | [Trial_Protocol(NEUT_OR_COND) == 1]
    (junction 355) -> swapCondBlock [order 3] : %if first cond block finished
        | [condCount == 1]
    neutEvents -> waitForHold1 : after(1,msec)
    conditionEvents -> nice1 : after(1,msec)
    Approached -> nice [order 1] : %approached cond2/neut2 during approach cond1/neut1 block
        | [(Trial_Protocol(TOGGLE_FIELD) == 1) && appAvoid == 0]
    Approached -> nice [order 2] : %approached cond1/neut1 during approach cond2/neut2 block
        | [(Trial_Protocol(TOGGLE_FIELD) == 0) && appAvoid == 1]
    locationEvents -> Approached [order 2] : %check if approached
        | e_approach
    nice -> checkError : after(1,msec)
    Approached -> success [order 3] : after(1,msec)
    nice1 -> loc1 [order 1] : %check where the
        | %target is
        | [appAngle == 1]
    nice1 -> loc2 [order 2] : [appAngle == 2]
    Avoided -> nice [order 1] : %avoided cond2/neut2 during an approach cond2/neut2 block
        | [(Trial_Protocol(TOGGLE_FIELD) == 1) && appAvoid == 1]
    checkError -> EndOfTrial : %delay after error trial
        | after(postRespDelay,msec)
    nice1 -> loc3 [order 3] : [appAngle == 3]
    locationEvents -> Avoided [order 3] : %check if avoided
        | e_avoid
    Avoided -> nice [order 2] : %avoided cond1/neut1 during an approach cond1/neut1 block
        | [(Trial_Protocol(TOGGLE_FIELD) == 0) && appAvoid == 0]
    nice1 -> loc4 [order 4] : [appAngle == 4]
    nice1 -> loc5 [order 5] : [appAngle == 5]
    Avoided -> success [order 3] : after(1,msec)
    nice1 -> loc6 [order 6] : [appAngle == 6]
    nice1 -> loc7 [order 7] : [appAngle == 7]
    nice1 -> loc8 [order 8] : [appAngle == 8]
    success -> EndOfTrial : %delay for success
        | after(postRespDelay,msec)
    nice1 -> loc9 [order 9] : [appAngle == 9]
    nice1 -> loc10 [order 10] : [appAngle == 10]
    nice1 -> loc11 [order 11] : [appAngle == 11]
    locationEvents -> TimedOut [order 1] : %delay for reaching to target
        | after(reachTO, msec)
    nice1 -> loc12 [order 12] : [appAngle == 12]
    TimedOut -> EndOfTrial : %delay after error trial
        | after(postRespDelay,msec)
  state Inter_Trial_State/
    %close all
    entry:
    event_code = 0;
    toggleField = 0; %turn off forcefield
    targetApp_state = 0; %turn off approach target
    targetStart_state = 0; %turn off start target
    targetAvoid_state = 0; %turn off avoid target
    targetLabel_state = 0; %turn off label
    repeat_trial_flag = 0;
    e_Trial_End;
  state RepeatTrial/
    repeat_trial_flag = 1;
  (junction 173) -> StartofTrial [order 1] : %keep the trials flowing if the block hasn't changed
      | [currentBlock == blockCheck]
  (default) -> Initialize
  Initialize -> outputBlockOrder : %wait for task to start
      | [currentTP > 0]
  (junction 173) -> (junction 323) [order 2] : %check if next block is different from last block
      | %so the TP counter and randomization resets if
      | %the block isnt the 2nd of 2 blocks because 2 blocks
      | %are needed to test approach and avoidance for both
      | %conditions or neutrals
      | [currentBlock ~= blockCheck]
  Inter_Trial_State -> (junction 173) : after(1,msec)
  RepeatTrial -> Inter_Trial_State : after(1,msec)
  MainTrial -> RepeatTrial : e_ExitTrialNow
  EndOfTrial -> Inter_Trial_State : after(1, msec)
  data: outLoc function_output; aRand function_input; bRand function_input; TPCount function_input; TPCurrent function_input; outCondNeut function_output; event_code output [0..]; repeat_trial_flag output; targetBegin_row output double; targetBegin_state output; targetLabel_row output; targetLabel_state output; targetInfo_row output; targetInfo_state output; targetStart_row output; targetStart_state output; targetAvoid_row output; targetAvoid_state output; targetApp_row output [1..32]; targetApp_state output; appAngle output; Trial_Protocol input; toggleField output; HandInTarget input; reachDelay input; reachRand input; reachTO input; postRespDelay input; startBlock input; currentBlock input; appAvoidNeut local; currentTP input; condCount local; appAvoidCond local; appAvoid local; randA local; randB local; blockCheck local; countTP local; randReach local; numTP local; condNeut local; neutCount local
  data targetApp_row settings: description=index of the row currently being used in the TargetTable
  events: e_clk input RISING_EDGE_EVENT; e_ExitTrialNow input RISING_EDGE_EVENT; e_Trial_End output EITHER_EDGE_EVENT; e_approach input EITHER_EDGE_EVENT; e_avoid input EITHER_EDGE_EVENT
  function [outLoc, outCondNeut] = arraySets(aRand,bRand,TPCount,TPCurrent):
    | function [outLoc, outCondNeut] = arraySets(aRand,bRand,TPCount,TPCurrent)
    | %This function sets up a pseudorandom order for the location of targets and
    | %which arm gets tested (numSpots must be set to 12 and numRows needs to 
    | %account for the number of trials, i think 16 is fine)
    | 
    | %% set up random arrays for location and arm
    | %Random arrays are generated that put each of the approach and avoid
    | %targets in 1 of 12 locations for each arm.
    | 
    | outLoc = 0; %where is the location
    | outCondNeut = 0;  %which condition is the trial? (1 = cond1, 2 = cond2, 3 = neut1, 4 = neut2)
    | TPTot = 24; %total TP
    | numLoc = 12; %number of locations
    | 
    | %assumed 24 TP with each TP having 6 images
    | activeImageTP = TPTot/4; %active images are TP1-6
    | sedenImageTP = TPTot/2; %seden images are TP7-12
    | circImageTP = TPTot*3/4; %circle images are TP13-18
    | squareImageTP = TPTot; %square images are TP19-24
    | 
    | allActive = sum(TPCount(1:activeImageTP)); %get the current number of active images trials completed
    | allSeden = sum(TPCount(activeImageTP+1:sedenImageTP)); %get the current number of seden images trials completed
    | allCirc = sum(TPCount(sedenImageTP+1:circImageTP)); %get the current number of circ images trials completed
    | allSqu = sum(TPCount(circImageTP+1:squareImageTP)); %get the current number of square images trials completed
    | 
    | if (TPCurrent <= activeImageTP) %current TP is active image
    |     outLoc = aRand(allActive); %access random value (1-12) to put new target based on current number of active image trials completed
    |     outCondNeut = 1;
    | elseif (TPCurrent > activeImageTP && TPCurrent <= sedenImageTP) %current TP is seden image
    |     outLoc = bRand(allSeden); %access random value (1-12) to put new target based on current number of seden image trials completed
    |     outCondNeut = 2;
    | elseif (TPCurrent > sedenImageTP && TPCurrent <= circImageTP) %current TP is circle image
    |     outLoc = aRand(allCirc); %access random value (1-12) to put new target based on current number of circle image trials completed
    |     outCondNeut = 3;
    | elseif (TPCurrent > circImageTP) %current TP is square image
    |     outLoc = bRand(allSqu); %access random value (1-12) to put new target based on current number of square image trials completed
    |     outCondNeut = 4;
    | end

== matlab function KinarmUAATask_260120/ForceField Controller/EP Force Controller ==
  data: TASK_WIDE input; MAX_FORCE parameter; forcesIn input; forcesOut output
function forcesOut  = fcn(TASK_WIDE, MAX_FORCE, forcesIn)
%Function applies a load to the arm to keep the hand away from a target
%and the trial is a loaded trial (toggleField == 1).
%acts as a deterent force but should be very small MAX_FORCE in Task Wide
%Parameters, currently set as 1 in the .dtp

%% initialize
maxForce = TASK_WIDE(MAX_FORCE); %amount of the forcefield

%% set forces out
%Send out forces to the appropriate arm.

posCon_force1 = sqrt(forcesIn(1)^2 + forcesIn(2)^2);
posCon_force2 = sqrt(forcesIn(3)^2 + forcesIn(4)^2);

forcesOut = -forcesIn;
% limit the force of arm 1
if posCon_force1 > maxForce
    scaling = maxForce / posCon_force1;
    forcesOut(1:2) = forcesOut(1:2) * scaling;
end

% limit the force of arm 2
if posCon_force2 > maxForce
    scaling = maxForce / posCon_force2;
    forcesOut(3:4) = forcesOut(3:4) * scaling;
end

== matlab function KinarmUAATask_260120/numberGenerator/taskWideInitialize ==
  data: TASK_WIDE input; reachDelay output; reachRand output; reachTO output; postRespDelay output; REACH_DELAY parameter; REACH_RAND parameter; REACH_TO parameter; POSTRESP_DELAY parameter; startBlock output; START_BLOCK parameter
function [reachDelay, reachRand, reachTO, postRespDelay, startBlock] =...
    fcn(TASK_WIDE, REACH_DELAY, REACH_RAND, REACH_TO, POSTRESP_DELAY, START_BLOCK)  

%% task wide parameter outputs
reachDelay = TASK_WIDE(REACH_DELAY); %time for holding hand in trial start target
reachRand = TASK_WIDE(REACH_RAND); %random time added to reachDelay
reachTO = TASK_WIDE(REACH_TO); %time to approach or avoid
postRespDelay = TASK_WIDE(POSTRESP_DELAY); %time between trials
startBlock = TASK_WIDE(START_BLOCK); %time to hold the start target to begin a block

== matlab function KinarmUAATask_260120/textMod/textMod ==
  data: textIn input; pickText input; textOut output
function textOut  = fcn(textIn, pickText)
%modify the label target to display text

textOut = textIn;
if (pickText == 1) %labeltarget state 1
    str1 = ['Keep your cursor in the circle to start'];
elseif (pickText == 2) %labeltarget state 2
    str1 = ['Incorrect!'];
elseif (pickText == 3) %labeltarget state 3
    str1 = ['Too slow!'];
else
    str1 = ' ';
end
textOut(1,15:(length(str1)+14))=uint16(str1);  %str in letters

== stateflow chart KinarmUAATask_260120/ForceField Controller/PaddleContact/Ramp_up_down ==
  state peak/
    entry:
    scaling=1;
  state RampingUp/
    %sigmoidal ramping taken from Ethan Heming and
    %modified by Kayne
    entry:
    tick=0;
    CurrScale=scaling;
    b=ramp/4; % Center at Middle;
    c=ramp/20; % Define Rise Rate;
    during:
    tick++;
    scaling = (1-CurrScale)/(1+exp(-1*(tick-b)/c))+CurrScale;
  state RampingDown/
    entry:
    tick=0;
    CurrScale=scaling;
    b=ramp/4; % Center at Middle;
    c=ramp/20; % Define Drop Rate;
    during:
    tick++;
    scaling = CurrScale*(1-1/(1+exp(-1*(tick-b)/c)));
  state minimum/
    entry:
    scaling=0;
  peak -> RampingDown [order 1] : %check if forcefield is turned off
      | [fieldOn == 0]
  RampingUp -> peak : after(ramp, e_clk)
  peak -> RampingDown [order 2] : %check if hand is outside target
      | [inRange == 0]
  RampingDown -> minimum : after(ramp, e_clk)
  minimum -> RampingUp : %check if hand is in target and
      | %trial has a forcefield
      | [inRange == 1 && fieldOn == 1]
  (default) -> minimum
  data: ramp input double; scaling output double; tick local double; c local double; b local double; CurrScale local double; inRange input double; fieldOn input double
  events: e_clk input RISING_EDGE_EVENT
